simulink model "quartercar_RL_6_no_G_last"  (R2023a)
settings: Solver=VariableStepAuto  StartTime=0  StopTime=10  FixedStep=0.05  RelTol=1e-5  EnableMultiTasking=on
model workspace (MAT data in the model file):
  cs = 2126
  ks = 24000
  kt = 243000
  ms = 365
  mu = 43
undefined symbols (not defined in the file or in its folder): magnitude
libraries: simulink x3, rllib x1
settings Model: Creator=Administrator  LastModifiedBy=Yuk
settings SolverCC: AllowMultiTaskInputOutput=on  InsertRTBMode=Never (minimum delay)
settings DataIOCC: SaveFormat=Array
settings OptimizationCC: LifeSpan=inf
settings DebuggingCC: AlgebraicLoopMsg=none  UnderspecifiedInitializationDetection=Classic  MergeDetectMultiDrivingBlocksExec=none  SolverPrmCheckMsg=warning  UnconnectedInputMsg=warning  UnconnectedOutputMsg=warning  UnconnectedLineMsg=warning  StateNameClashWarn=warning  SFUnexpectedBacktrackingDiag=warning  SFNoUnconditionalDefaultTransitionDiag=warning  SFExecutionAtInitializationDiag=none  ArithmeticOperatorsInVariantConditions=warning
settings HardwareCC: ProdBitPerPointer=32  ProdBitPerSizeT=32  ProdBitPerPtrDiffT=32  ProdLargestAtomicFloat=None  ProdIntDivRoundTo=Undefined  ProdEndianess=Unspecified  ProdWordSize=32  ProdHWDeviceType=32-bit Generic
settings ModelReferenceCC: PropagateSignalLabelsOutOfModel=off
settings SFSimCC: SimUseLocalCustomCode=off  CustomCodeUndefinedFunction=UseInterfaceOnly  SimTargetLang=C++
settings RTWCC: RTWUseLocalCustomCode=off
settings CodeAppCC: StateflowObjectComments=on
settings GRTTargetCC: TargetLangStandard=C89/C90 (ANSI)
settings ConfigComp: CovMetricSettings=dw  CovSaveCumulativeToWorkspaceVar=on  CovSaveSingleToWorkspaceVar=on  CovExternalEMLEnable=off

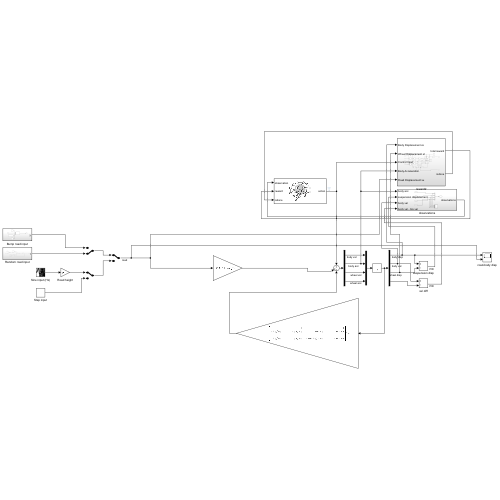
[thumbnail: Simulink's stored preview of the top-level diagram]
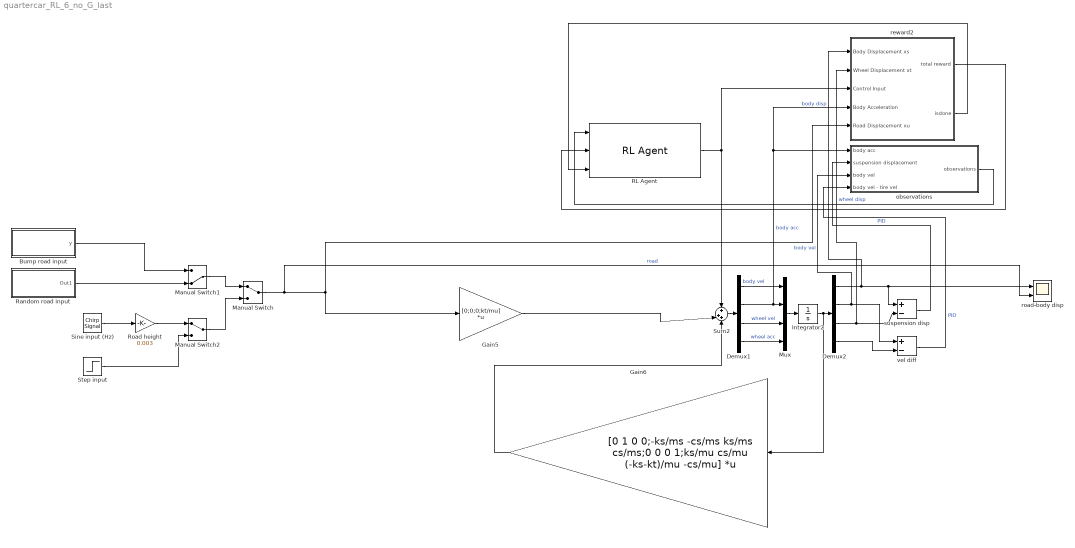
== system quartercar_RL_6_no_G_last ==
  Bump road input : Subsystem
  Demux1 : Demux
  Demux2 : Demux
  Gain5 : Gain  Gain=[0;0;0;kt/mu]  Multiplication=Matrix(K*u)
  Gain6 : Gain  Gain=[0 1 0 0;-ks/ms -cs/ms ks/ms cs/ms;0 0 0 1;ks/mu cs/mu (-ks-kt)/mu -cs/mu]  Multiplication=Matrix(K*u)
  Integrator2 : Integrator
  Manual Switch : ManualSwitch
  Manual Switch1 : ManualSwitch  CurrentSetting=0
  Manual Switch2 : ManualSwitch
  Mux : Mux
  RL Agent : rllib/RL Agent  Agent=saved_agent  ExternalActionAsInput=off  ProvideLastAction=off  ProvideCumRwd=off  TreatAsDirectFeedthrough=on  UseStrictObservationDataTypes=off
  Random road input : Subsystem
  Road height : Gain  Gain=0.003
  Sine input (Hz) : simulink/Sources/Chirp Signal  f1=1  T=10  f2=1
  Step input : Step  SampleTime=0
  Sum2 : Sum  Inputs=+|++
  observations : Subsystem
  reward2 : Subsystem
  road-body disp : Scope  NumInputPorts=2
  suspension disp : Sum  Inputs=+-
  vel diff : Sum  Inputs=+-
  wires:
  Gain6/1 -> Sum2/3
  Sum2/1 -> Demux1/1
  Demux2/1 -> reward2/1(Body Displacement xs), road-body disp/1, suspension disp/1  "body disp"
  Demux2/3 -> reward2/2(Wheel Displacement xt), suspension disp/2  "wheel disp"
  Gain5/1 -> Sum2/2
  Manual Switch/1 -> road-body disp/2, Gain5/1, reward2/5(Road Displacement xu)  "road"
  Integrator2/1 -> Gain6/1, Demux2/1
  Demux1/1 -> Mux/1  "body vel"
  Demux1/2 -> reward2/4(Body Acceleration), observations/1(body acc), Mux/2  "body acc"
  Demux1/3 -> Mux/3  "wheel vel"
  Demux1/4 -> Mux/4  "wheel acc"
  Mux/1 -> Integrator2/1
  Bump road input/1(y) -> Manual Switch1/1
  Random road input/1(Out1) -> Manual Switch1/2
  Sine input (Hz)/1 -> Road height/1
  Step input/1 -> Manual Switch2/2
  Manual Switch1/1 -> Manual Switch/1
  Manual Switch2/1 -> Manual Switch/2
  Road height/1 -> Manual Switch2/1
  observations/1(observations) -> RL Agent/1
  RL Agent/1 -> reward2/3(Control Input), Sum2/1
  reward2/1(total reward) -> RL Agent/2
  reward2/2(isdone) -> RL Agent/3
  suspension disp/1 -> observations/2(suspension displacement)  "PID"
  Demux2/2 -> observations/3(body vel), vel diff/1  "body vel"
  Demux2/4 -> vel diff/2
  vel diff/1 -> observations/4(body vel - tire vel)  "PID"

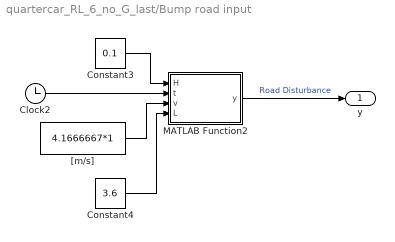
== system quartercar_RL_6_no_G_last/Bump road input ==
  Clock2 : Clock
  Constant3 : Constant  Value=0.1
  Constant4 : Constant  Value=3.6
  MATLAB Function2 : MATLAB Function  TreatAsAtomicUnit=on
  "[m/s]" : Constant  Value=4.1666667*1
  y : Outport
  wires:
  Clock2/1 -> MATLAB Function2/2(t)
  Constant4/1 -> MATLAB Function2/4(L)
  MATLAB Function2/1(y) -> y/1  "Road Disturbance"
  Constant3/1 -> MATLAB Function2/1(H)
  "[m/s]"/1 -> MATLAB Function2/3(v)

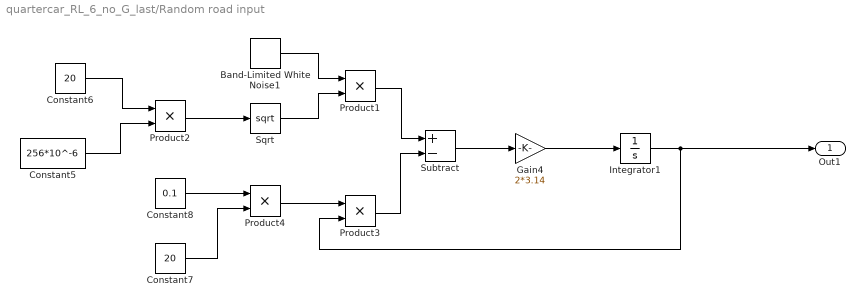
== system quartercar_RL_6_no_G_last/Random road input ==
  Band-Limited White Noise1 : simulink/Sources/Band-Limited White Noise  Cov=[5.4*10^-3]  Ts=0.1  seed=[23341]
  Constant5 : Constant  Value=256*10^-6
  Constant6 : Constant  Value=20
  Constant7 : Constant  Value=20
  Constant8 : Constant  Value=0.1
  Gain4 : Gain  Gain=2*3.14
  Integrator1 : Integrator
  Product{1..4} (4 alike) : Product
  Sqrt : Sqrt
  Subtract : Sum  Inputs=+-
  Out1 : Outport
  wires:
  Subtract/1 -> Gain4/1
  Product2/1 -> Sqrt/1
  Constant8/1 -> Product4/1
  Constant7/1 -> Product4/2
  Product4/1 -> Product3/1
  Constant6/1 -> Product2/1
  Gain4/1 -> Integrator1/1
  Integrator1/1 -> Product3/2, Out1/1
  Product1/1 -> Subtract/1
  Band-Limited White Noise1/1 -> Product1/1
  Product3/1 -> Subtract/2
  Sqrt/1 -> Product1/2
  Constant5/1 -> Product2/2

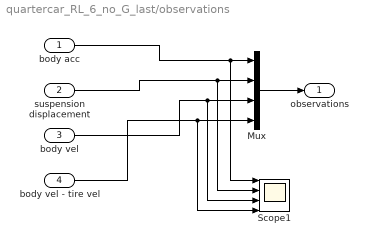
== system quartercar_RL_6_no_G_last/observations ==
  body acc : Inport
  suspension displacement : Inport  Port=2
  body vel : Inport  Port=3
  body vel - tire vel : Inport  Port=4
  Mux : Mux
  Scope1 : Scope  NumInputPorts=4
  observations : Outport
  wires:
  body acc/1 -> Scope1/1, Mux/1
  Mux/1 -> observations/1
  body vel/1 -> Scope1/3, Mux/3
  suspension displacement/1 -> Scope1/2, Mux/2
  body vel - tire vel/1 -> Scope1/4, Mux/4

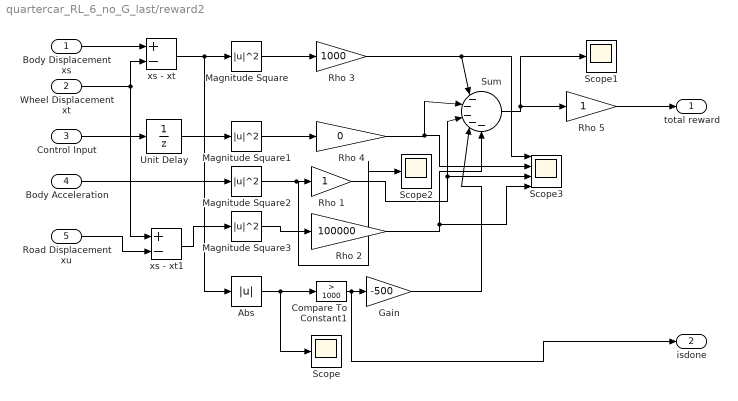
== system quartercar_RL_6_no_G_last/reward2 ==
  Body Displacement xs : Inport
  Wheel Displacement xt : Inport  Port=2
  Control Input : Inport  Port=3
  Body Acceleration : Inport  Port=4
  Road Displacement xu : Inport  Port=5
  Abs : Abs  SaturateOnIntegerOverflow=off
  Compare To Constant1 : simulink/Logic and Bit Operations/Compare To Constant  relop=>  const=1000  OutDataTypeStr=boolean
  Gain : Gain  Gain=-500
  Magnitude Square{,1..3} (4 alike) : Math  Operator=magnitude^2  SignedPower=on  RndMeth=Zero
  Rho 1 : Gain
  Rho 2 : Gain  Gain=100000
  Rho 3 : Gain  Gain=1000
  Rho 4 : Gain  Gain=0
  Rho 5 : Gain
  Scope : Scope
  Scope1 : Scope
  Scope2 : Scope
  Scope3 : Scope  NumInputPorts=4
  Sum : Sum  Inputs=|-----
  Unit Delay : UnitDelay  SampleTime=-1  HasFrameUpgradeWarning=on
  xs - xt : Sum  Inputs=+-
  xs - xt1 : Sum  Inputs=+-
  total reward : Outport
  isdone : Outport  Port=2
  wires:
  Wheel Displacement xt/1 -> xs - xt1/1, xs - xt/2
  Body Displacement xs/1 -> xs - xt/1
  Magnitude Square2/1 -> Scope2/1, Rho 1/1
  xs - xt/1 -> Magnitude Square/1, Abs/1
  Magnitude Square/1 -> Rho 3/1
  Control Input/1 -> Unit Delay/1
  Unit Delay/1 -> Magnitude Square1/1
  Rho 3/1 -> Scope3/1, Sum/1
  Sum/1 -> Rho 5/1, Scope1/1
  Compare To Constant1/1 -> isdone/1, Gain/1
  Rho 1/1 -> Scope3/3, Sum/3
  Gain/1 -> Sum/4
  Body Acceleration/1 -> Magnitude Square2/1
  Rho 5/1 -> total reward/1
  Abs/1 -> Scope/1, Compare To Constant1/1
  Rho 4/1 -> Scope3/2, Sum/2
  Magnitude Square1/1 -> Rho 4/1
  Road Displacement xu/1 -> xs - xt1/2
  xs - xt1/1 -> Magnitude Square3/1
  Magnitude Square3/1 -> Rho 2/1
  Rho 2/1 -> Scope3/4, Sum/5

== matlab function quartercar_RL_6_no_G_last/Bump road input/MATLAB Function2 ==
  data: H input; y output; t input; v input; L input
function y = fcn(H,t,v,L)
% CODE GENERATION
if (0.5<t) && (t<L/v+0.5)
    
  y=H/2*(1-cos((2*pi*v/L)*(t-0.5)));
% w = 2*pi*v/L;
%   y=H*(1-cos(w*t));

else
    y=0;
end
out=y;
